simulink model "sm_car_Axle3_withDSD"  (R2022a)
settings: Solver=ode23t  StartTime=0.0  StopTime=40  MaxStep=0.4  RelTol=1e-3  AbsTol=1e-3  EnableMultiTasking=on
PreLoadFcn:
  | disp('Loading default data for 3-axle vehicle and 2-axle trailer')
  | if verLessThan('matlab', '9.11')
  |     load Vehicle_Axle3_008
  |     Vehicle = Vehicle_Axle3_008;
  |     load Trailer_Axle2_000
  |     Trailer = Trailer_Axle2_000;
  | else
  |     load Vehicle_Axle3_019
  |     Vehicle = Vehicle_Axle3_019;
  |     load Trailer_Axle2_022
  |     Trailer = Trailer_Axle2_022;
  | end
  | 
  | disp('Turning off MFEval warnings...')
  | disp('Solver:CoeffChecks:Eyk -- OFF')
  | disp('Solver:Limits:Exceeded -- OFF')
  | disp('Solver:CoeffChecks:Et -- OFF')
  | disp('Solver:CoeffChecks:Exa -- OFF')
  | 
  | warning('off','Solver:CoeffChecks:Eyk')
  | warning('off','Solver:Limits:Exceeded')
  | warning('off','Solver:CoeffChecks:Et')
  | warning('off','Solver:CoeffChecks:Exa')
  | %warning('off','Solver:Radius:NegativeRho')
  | 
  | % Due to usability issue in Repeating Sequence block
  | warning('off','Simulink:Masking:Invalid');
  | 
  | % Eliminate unnecessary warnings in inactive variants
  | % Warnings generated only if you click through inactive variant
  | warning('off','MATLAB:nonExistentField');
  | warning('off','Simulink:Parameters:BlkParamUndefined');
PostLoadFcn:
  | set_param([bdroot '/Vehicle'],'popup_trailer','On')
  | warning('off','sm:sli:setup:compile:LocalSolverNotSupported')
  | sm_car_config_maneuver(bdroot,'WOT Braking');
  | sm_car_config_vehicle(bdroot,false);
  | sm_car_config_logging(bdroot);
InitFcn:
  | sm_car_config_camera;
  | Vehicle = sm_car_vehcfg_checkConfig(Vehicle);
StartFcn:
  | sm_car_check_tire_model(bdroot);
  | tic;
StopFcn:
  | Elapsed_Sim_Time = toc;
  | % disp(['Elapsed Sim Time = ' num2str(Elapsed_Sim_Time)]);
values from neighbouring files (symbols this model uses):
  scenario = drivingScenario    [AEB_PedestrianChild_Nearside_50width_overrun.m]
undefined symbols (not defined in the file or in its folder): Maneuver, SimParams, X, Y, Z
libraries: simulink x16, Tire_Utilities x7, sm_lib x6, sm_car_DSD_lib x3, World_Config_Utilities x2, Maneuver_Get_Pose x2, Vehicle_Visualization x2, drivingscenarioandsensors x1, Camera_Frame_Definitions x1, Brake_Control x1, Driveline_Control_Axle2_None x1, Power_Control_Axle2_FixedRatio x1
(part 1 of 3)
CloseFcn:
  | try,close(h1_sm_car),end
  | clear h1_sm_car
  | try,close(h2_sm_car),end
  | clear h2_sm_car
  | try,close(h3_sm_car),end
  | clear h3_sm_car
  | try,close(h4_sm_car),end
  | clear h4_sm_car
  | 
  | 
  | clear simlog_sm_car
  | clear logsout_sm_car
Description:
  | Full Vehicle with Multibody Suspension
  | 
  | Copyright 2018-2024 The MathWorks, Inc.
settings Model: Creator=smiller  LastModifiedBy=smiller
settings SolverCC: ConcurrentTasks=on  AlgebraicLoopSolver=TrustRegion  AutoInsertRateTranBlk=on  InsertRTBMode=Never (minimum delay)
settings DataIOCC: MaxDataPoints=10000  SaveFormat=StructureWithTime  ReturnWorkspaceOutputs=off  SignalLoggingName=logsout_sm_car
settings OptimizationCC: BlockReduction=off  OptimizeBlockIOStorage=off  BufferReuse=off  GlobalBufferReuse=off  ExpressionFolding=off  LocalBlockOutputs=off  OptimizeDataStoreBuffers=off  BusAssignmentInplaceUpdate=off
settings DebuggingCC: ParameterPrecisionLossMsg=none  UnconnectedInputMsg=warning  UnconnectedOutputMsg=warning  UnconnectedLineMsg=warning  ArithmeticOperatorsInVariantConditions=warning
settings HardwareCC: ProdBitPerPointer=32  ProdBitPerSizeT=32  ProdBitPerPtrDiffT=32  ProdLargestAtomicFloat=None  ProdWordSize=32  ProdLongLongMode=on  ProdHWDeviceType=Generic->32-bit x86 compatible
settings SFSimCC: CustomCodeUndefinedFunction=UseInterfaceOnly
settings RTWCC: Description=Generic Real-Time Target  DLArmComputeVersion=19.05
settings GRTTargetCC: TargetLangStandard=C89/C90 (ANSI)
settings SimscapeCC: SimscapeLogType=all  SimscapeLogSimulationStatistics=on  SimscapeLogName=simlog_sm_car  SimscapeLogDataHistory=100000  SimscapeOperatingPoint=ssc_op
settings DiagnosticsConfigSet: SimMechanicsConflictingReferenceFrames=none  SimMechanicsRigidlyBoundBlock=none  SimMechanicsUnsatisfiedHighPriorityTargets=error
settings ExplorerConfigSet: InternalSimMechanicsExplorerSettings="<ExplorerConfiguration><canonicalview>default</canonicalview><AnimationSetting><BasePlaybackSpeed>1.0</BasePlaybackSpeed><PlaybackSpeedFactor>2.0</PlaybackSpeedFactor></AnimationSetting><TilePanel><TileInfo><Tiles Columns=\"2\" Count=\"2\" Rows=\"1\"><Column Weight=\"0.6237\"/><Column Weight=\"0.3763\"/><Row Weight=\"1\"/><Tile Height=\"1\" Width=\"1\" X=\"0\" Y=\"0\"/><Tile Height=\"1\" Width=\"1\" X=\"1\" Y=\"0\"/></Tiles></TileInfo><SceneInfo><SceneViewer><BGColor><R>1</R><G>1</G><B>1</B></BGColor><Camera><DoPerspective>on</DoPerspective><Position><X>30.8247101063582534</X><Y>0.571181504346149893</Y><Z>2.94604477699006129</Z></Position><Center><X>31.8244257672194557</X><Y>0.571174262025495705</Y><Z>2.92219949702943582</Z></Center><Up><X>0.0238451835733496931</X><Y>0.00316311256438651369</Y><Z>0.999710659110554012</Z></Up><ViewLimDist>1</ViewLimDist><YLim>0.466307658154998583</YLim><XLim>0.468997894644354318</XLim></Camera></SceneViewer><SceneViewer><BGColor><R>1</R><G>1</G><B>1</B></BGColor><Camera><DoPerspective>off</DoPerspective><Position><X>19.6858043140873598</X><Y>0.0564739167979380133</Y><Z>285.626212837348305</Z></Position><Center><X>19.6858043140873598</X><Y>0.0564739167979380133</Y><Z>2.09091177841753506</Z></Center><Up><X>0.999998132884981517</X><Y>0.0019324146943363596</Y><Z>0</Z></Up><ViewLimDist>1</ViewLimDist><YLim>18.8750577870123131</YLim><XLim>11.3976310483112808</XLim></Camera></SceneViewer></SceneInfo></TilePanel><MechEditorPanel><Cameras><Camera><Id>Camera1</Id><Value><Name>Track FixO FR</Name><NativeCamera><PositionTrackingFeature>Camera_Frames.Frame_FixO_FR.R</PositionTrackingFeature><CenterTrackingFeature>Camera_Frames.Frame_FixO_FR.R</CenterTrackingFeature><UpVectorTrackingFeature>Camera_Frames.Frame_FixO_FR.R</UpVectorTrackingFeature><CenterTrackingOrigin>off</CenterTrackingOrigin><CenterTrackingDirection>+X</CenterTrackingDirection><UpVectorTrackingDirection>+Z</UpVectorTrackingDirection></NativeCamera></Value></Camera><Camera><Id>Camera2</Id><Value><Name>Track FixO Right</Name><NativeCamera><PositionTrackingFeature>Camera_Frames.Frame_FixO_Right.R</PositionTrackingFeature><CenterTrackingFeature>Camera_Frames.Transform_Camera_Ref.F</CenterTrackingFeature><UpVectorTrackingFeature>Camera_Frames.Frame_FixO_Right.R</UpVectorTrackingFeature><CenterTrackingOrigin>off</CenterTrackingOrigin><CenterTrackingDirection>+Y</CenterTrackingDirection><UpVectorTrackingDirection>+Z</UpVectorTrackingDirection></NativeCamera></Value></Camera><Camera><Id>Camera3</Id><Value><Name>Track FixO RR</Name><NativeCamera><PositionTrackingFeature>Camera_Frames.Frame_FixO_RR.R</PositionTrackingFeature><CenterTrackingFeature>Camera_Frames.Frame_FixO_RR.R</CenterTrackingFeature><UpVectorTrackingFeature>Camera_Frames.Frame_FixO_RR.R</UpVectorTrackingFeature><CenterTrackingOrigin>off</CenterTrackingOrigin><CenterTrackingDirection>+X</CenterTrackingDirection><UpVectorTrackingDirection>+Z</UpVectorTrackingDirection></NativeCamera></Value></Camera><Camera><Id>Camera4</Id><Value><Name>Track FixO RL</Name><NativeCamera><PositionTrackingFeature>Camera_Frames.Frame_FixO_RL.R</PositionTrackingFeature><CenterTrackingFeature>Camera_Frames.Frame_FixO_RL.R</CenterTrackingFeature><UpVectorTrackingFeature>Camera_Frames.Frame_FixO_RL.R</UpVectorTrackingFeature><CenterTrackingOrigin>off</CenterTrackingOrigin><CenterTrackingDirection>+X</CenterTrackingDirection><UpVectorTrackingDirection>+Z</UpVectorTrackingDirection></NativeCamera></Value></Camera><Camera><Id>Camera5</Id><Value><Name>Track FixO Left</Name><NativeCamera><PositionTrackingFeature>Camera_Frames.Frame_FixO_Left.R</PositionTrackingFeature><CenterTrackingFeature>Camera_Frames.Transform_Camera_Ref.F</CenterTrackingFeature><UpVectorTrackingFeature>Camera_Frames.Frame_FixO_Left.R</UpVectorTrackingFeature><CenterTrackingOrigin>off</CenterTrackingOrigin><CenterTrackingDirection>-Y</CenterTrackingDirection><UpVectorTrackingDirection>+Z</UpVectorTrackingDirection></NativeCamera></Value></Camera><Camera><Id>Camera6</Id><Value><Name>Track FixO FL</Name><NativeCamera><PositionTrackingFeature>Camera_Frames.Frame_FixO_FL.R</PositionTrackingFeature><CenterTrackingFeature>Camera_Frames.Frame_FixO_FL.R</CenterTrackingFeature><UpVectorTrackingFeature>Camera_Frames.Frame_FixO_FL.R</UpVectorTrackingFeature><CenterTrackingOrigin>off</CenterTrackingOrigin><CenterTrackingDirection>+X</CenterTrackingDirection><UpVectorTrackingDirection>+Z</UpVectorTrackingDirection></NativeCamera></Value></Camera><Camera><Id>Camera7</Id><Value><Name>Track FixO Top</Name><NativeCamera><PositionTrackingFeature>Camera_Frames.Frame_FixO_Top.R</PositionTrackingFeature><CenterTrackingFeature>Camera_Frames.Frame_FixO_Top.R</CenterTrackingFeature><UpVectorTrackingFeature>Camera_Frames.Frame_FixO_Top.R</UpVectorTrackingFeature><CenterTrackingOrigin>off</CenterTrackingOrigin><CenterTrackingDirection>+X</CenterTrackingDirection><UpVectorTrackingDirection>+Z</UpVectorTrackingDirection></NativeCamera></Value></Camera><Camera><Id>Camera8</Id><Value><Name>Track FixO Front</Name><NativeCamera><PositionTrackingFeature>Camera_Frames.Frame_FixO_Front.R</PositionTrackingFeature><CenterTrackingFeature>Camera_Frames.Frame_FixO_Front.R</CenterTrackingFeature><UpVectorTrackingFeature>Camera_Frames.Frame_FixO_Front.R</UpVectorTrackingFeature><CenterTrackingOrigin>off</CenterTrackingOrigin><CenterTrackingDirection>+X</CenterTrackingDirection><UpVectorTrackingDirection>+Z</UpVectorTrackingDirection></NativeCamera></Value></Camera><Camera><Id>Camera9</Id><Value><Name>Track FixO Rear</Name><NativeCamera><PositionTrackingFeature>Camera_Frames.Frame_FixO_Rear.R</PositionTrackingFeature><CenterTrackingFeature>Camera_Frames.Frame_FixO_Rear.R</CenterTrackingFeature><UpVectorTrackingFeature>Camera_Frames.Frame_FixO_Rear.R</UpVectorTrackingFeature><CenterTrackingOrigin>off</CenterTrackingOrigin><CenterTrackingDirection>+X</CenterTrackingDirection><UpVectorTrackingDirection>+Z</UpVectorTrackingDirection></NativeCamera></Value></Camera><Camera><Id>Camera10</Id><Value><Name>Track FR</Name><NativeCamera><PositionTrackingFeature>Camera_Frames.Frame_FR.R</PositionTrackingFeature><CenterTrackingFeature>Camera_Frames.Frame_FR.R</CenterTrackingFeature><UpVectorTrackingFeature>Camera_Frames.Frame_FR.R</UpVectorTrackingFeature><CenterTrackingOrigin>off</CenterTrackingOrigin><CenterTrackingDirection>+X</CenterTrackingDirection><UpVectorTrackingDirection>+Z</UpVectorTrackingDirection></NativeCamera></Value></Camera><Camera><Id>Camera11</Id><Value><Name>Track Right</Name><NativeCamera><PositionTrackingFeature>Camera_Frames.Frame_Right.R</PositionTrackingFeature><CenterTrackingFeature>Camera_Frames.Transform_Camera_Ref.F</CenterTrackingFeature><UpVectorTrackingFeature>Camera_Frames.Frame_Right.R</UpVectorTrackingFeature><CenterTrackingOrigin>off</CenterTrackingOrigin><CenterTrackingDirection>+Y</CenterTrackingDirection><UpVectorTrackingDirection>+Z</UpVectorTrackingDirection></NativeCamera></Value></Camera><Camera><Id>Camera12</Id><Value><Name>Track RR</Name><NativeCamera><PositionTrackingFeature>Camera_Frames.Frame_RR.R</PositionTrackingFeature><CenterTrackingFeature>Camera_Frames.Frame_RR.R</CenterTrackingFeature><UpVectorTrackingFeature>Camera_Frames.Frame_RR.R</UpVectorTrackingFeature><CenterTrackingOrigin>off</CenterTrackingOrigin><CenterTrackingDirection>+X</CenterTrackingDirection><UpVectorTrackingDirection>+Z</UpVectorTrackingDirection></NativeCamera></Value></Camera><Camera><Id>Camera13</Id><Value><Name>Track RL</Name><NativeCamera><PositionTrackingFeature>Camera_Frames.Frame_RL.R</PositionTrackingFeature><CenterTrackingFeature>Camera_Frames.Frame_RL.R</CenterTrackingFeature><UpVectorTrackingFeature>Camera_Frames.Frame_RL.R</UpVectorTrackingFeature><CenterTrackingOrigin>off</CenterTrackingOrigin><CenterTrackingDirection>+X</CenterTrackingDirection><UpVectorTrackingDirection>+Z</UpVectorTrackingDirection></NativeCamera></Value></Camera><Camera><Id>Camera14</Id><Value><Name>Track Left</Name><NativeCamera><PositionTrackingFeature>Camera_Frames.Frame_Left.R</PositionTrackingFeature><CenterTrackingFeature>Camera_Frames.Transform_Camera_Ref.F</CenterTrackingFeature><UpVectorTrackingFeature>Camera_Frames.Frame_Left.R</UpVectorTrackingFeature><CenterTrackingOrigin>off</CenterTrackingOrigin><CenterTrackingDirection>-Y</CenterTrackingDirection><UpVectorTrackingDirection>+Z</UpVectorTrackingDirection></NativeCamera></Value></Camera><Camera><Id>Camera15</Id><Value><Name>Track FL</Name><NativeCamera><PositionTrackingFeature>Camera_Frames.Frame_FL.R</PositionTrackingFeature><CenterTrackingFeature>Camera_Frames.Frame_FL.R</CenterTrackingFeature><UpVectorTrackingFeature>Camera_Frames.Frame_FL.R</UpVectorTrackingFeature><CenterTrackingOrigin>off</CenterTrackingOrigin><CenterTrackingDirection>+X</CenterTrackingDirection><UpVectorTrackingDirection>+Z</UpVectorTrackingDirection></NativeCamera></Value></Camera><Camera><Id>Camera16</Id><Value><Name>Track Top</Name><NativeCamera><PositionTrackingFeature>Camera_Frames.Frame_Top.R</PositionTrackingFeature><CenterTrackingFeature>Camera_Frames.Frame_Top.R</CenterTrackingFeature><UpVectorTrackingFeature>Camera_Frames.Frame_Top.R</UpVectorTrackingFeature><CenterTrackingOrigin>off</CenterTrackingOrigin><CenterTrackingDirection>+X</CenterTrackingDirection><UpVectorTrackingDirection>+Z</UpVectorTrackingDirection></NativeCamera></Value></Camera><Camera><Id>Camera17</Id><Value><Name>Track Front</Name><NativeCamera><PositionTrackingFeature>Camera_Frames.Frame_Front.R</PositionTrackingFeature><CenterTrackingFeature>Camera_Frames.Frame_Front.R</CenterTrackingFeature><UpVectorTrackingFeature>Camera_Frames.Frame_Front.R</UpVectorTrackingFeature><CenterTrackingOrigin>off</CenterTrackingOrigin><CenterTrackingDirection>+X</CenterTrackingDirection><UpVectorTrackingDirection>+Z</UpVectorTrackingDirection></NativeCamera></Value></Camera><Camera><Id>Camera18</Id><Value><Name>Track Rear</Name><NativeCamera><PositionTrackingFeature>Camera_Frames.Frame_Rear.R</PositionTrackingFeature><CenterTrackingFeature>Camera_Frames.Frame_Rear.R</CenterTrackingFeature><UpVectorTrackingFeature>Camera_Frames.Frame_Rear.R</UpVectorTrackingFeature><CenterTrackingOrigin>off</CenterTrackingOrigin><CenterTrackingDirection>+X</CenterTrackingDirection><UpVectorTrackingDirection>+Z</UpVectorTrackingDirection></NativeCamera></Value></Camera><Camera><Id>Camera19</Id><Value><Name>Track SuspF</Name><NativeCamera><PositionTrackingFeature>Camera_Frames.Frame_SuspF.R</PositionTrackingFeature><CenterTrackingFeature>Camera_Frames.Frame_SuspF.R</CenterTrackingFeature><UpVectorTrackingFeature>Camera_Frames.Frame_SuspF.R</UpVectorTrackingFeature><CenterTrackingOrigin>off</CenterTrackingOrigin><CenterTrackingDirection>+X</CenterTrackingDirection><UpVectorTrackingDirection>+Z</UpVectorTrackingDirection></NativeCamera></Value></Camera><Camera><Id>Camera20</Id><Value><Name>Track SuspR</Name><NativeCamera><PositionTrackingFeature>Camera_Frames.Frame_SuspR.R</PositionTrackingFeature><CenterTrackingFeature>Camera_Frames.Frame_SuspR.R</CenterTrackingFeature><UpVectorTrackingFeature>Camera_Frames.Frame_SuspR.R</UpVectorTrackingFeature><CenterTrackingOrigin>off</CenterTrackingOrigin><CenterTrackingDirection>+X</CenterTrackingDirection><UpVectorTrackingDirection>+Z</UpVectorTrackingDirection></NativeCamera></Value></Camera><Camera><Id>Camera21</Id><Value><Name>Track WheelFR</Name><NativeCamera><PositionTrackingFeature>Camera_Frames.Frame_Wheel_FR.R</PositionTrackingFeature><CenterTrackingFeature>Camera_Frames.Frame_Wheel_FR.R</CenterTrackingFeature><UpVectorTrackingFeature>Camera_Frames.Frame_Wheel_FR.R</UpVectorTrackingFeature><CenterTrackingOrigin>off</CenterTrackingOrigin><CenterTrackingDirection>+X</CenterTrackingDirection><UpVectorTrackingDirection>+Z</UpVectorTrackingDirection></NativeCamera></Value></Camera><Camera><Id>Camera22</Id><Value><Name>Track WheelRR</Name><NativeCamera><PositionTrackingFeature>Camera_Frames.Frame_Wheel_RR.R</PositionTrackingFeature><CenterTrackingFeature>Camera_Frames.Frame_Wheel_RR.R</CenterTrackingFeature><UpVectorTrackingFeature>Camera_Frames.Frame_Wheel_RR.R</UpVectorTrackingFeature><CenterTrackingOrigin>off</CenterTrackingOrigin><CenterTrackingDirection>+X</CenterTrackingDirection><UpVectorTrackingDirection>+Z</UpVectorTrackingDirection></NativeCamera></Value></Camera><Camera><Id>Camera23</Id><Value><Name>Track WheelRL</Name><NativeCamera><PositionTrackingFeature>Camera_Frames.Frame_Wheel_RL.R</PositionTrackingFeature><CenterTrackingFeature>Camera_Frames.Frame_Wheel_RL.R</CenterTrackingFeature><UpVectorTrackingFeature>Camera_Frames.Frame_Wheel_RL.R</UpVectorTrackingFeature><CenterTrackingOrigin>off</CenterTrackingOrigin><CenterTrackingDirection>+X</CenterTrackingDirection><UpVectorTrackingDirection>+Z</UpVectorTrackingDirection></NativeCamera></Value></Camera><Camera><Id>Camera24</Id><Value><Name>Track WheelFL</Name><NativeCamera><PositionTrackingFeature>Camera_Frames.Frame_Wheel_FL.R</PositionTrackingFeature><CenterTrackingFeature>Camera_Frames.Frame_Wheel_FL.R</CenterTrackingFeature><UpVectorTrackingFeature>Camera_Frames.Frame_Wheel_FL.R</UpVectorTrackingFeature><CenterTrackingOrigin>off</CenterTrackingOrigin><CenterTrackingDirection>+X</CenterTrackingDirection><UpVectorTrackingDirection>+Z</UpVectorTrackingDirection></NativeCamera></Value></Camera><Camera><Id>Camera25</Id><Value><Name>View Seat FL</Name><NativeCamera><PositionTrackingFeature>Camera_Frames.Frame_View_Seat_FL.R</PositionTrackingFeature><CenterTrackingFeature>Camera_Frames.Frame_View_Seat_FL.R</CenterTrackingFeature><UpVectorTrackingFeature>Camera_Frames.Frame_View_Seat_FL.R</UpVectorTrackingFeature><CenterTrackingOrigin>off</CenterTrackingOrigin><CenterTrackingDirection>+X</CenterTrackingDirection><UpVectorTrackingDirection>+Z</UpVectorTrackingDirection></NativeCamera></Value></Camera><Camera><Id>Camera26</Id><Value><Name>View Seat FR</Name><NativeCamera><PositionTrackingFeature>Camera_Frames.Frame_View_Seat_FR.R</PositionTrackingFeature><CenterTrackingFeature>Camera_Frames.Frame_View_Seat_FR.R</CenterTrackingFeature><UpVectorTrackingFeature>Camera_Frames.Frame_View_Seat_FR.R</UpVectorTrackingFeature><CenterTrackingOrigin>off</CenterTrackingOrigin><CenterTrackingDirection>+X</CenterTrackingDirection><UpVectorTrackingDirection>+Z</UpVectorTrackingDirection></NativeCamera></Value></Camera><Camera><Id>Camera27</Id><Value><Name>View Susp FR</Name><NativeCamera><PositionTrackingFeature>Camera_Frames.Frame_View_Susp_FR.R</PositionTrackingFeature><CenterTrackingFeature>Camera_Frames.Frame_View_Susp_FR.R</CenterTrackingFeature><UpVectorTrackingFeature>Camera_Frames.Frame_View_Susp_FR.R</UpVectorTrackingFeature><CenterTrackingOrigin>off</CenterTrackingOrigin><CenterTrackingDirection>+X</CenterTrackingDirection><UpVectorTrackingDirection>+Z</UpVectorTrackingDirection></NativeCamera></Value></Camera><Camera><Id>Camera28</Id><Value><Name>View Susp RR</Name><NativeCamera><PositionTrackingFeature>Camera_Frames.Frame_View_Susp_RR.R</PositionTrackingFeature><CenterTrackingFeature>Camera_Frames.Frame_View_Susp_RR.R</CenterTrackingFeature><UpVectorTrackingFeature>Camera_Frames.Frame_View_Susp_RR.R</UpVectorTrackingFeature><CenterTrackingOrigin>off</CenterTrackingOrigin><CenterTrackingDirection>+X</CenterTrackingDirection><UpVectorTrackingDirection>+Z</UpVectorTrackingDirection></NativeCamera></Value></Camera><Camera><Id>Camera29</Id><Value><Name>View Susp RL</Name><NativeCamera><PositionTrackingFeature>Camera_Frames.Frame_View_Susp_RL.R</PositionTrackingFeature><CenterTrackingFeature>Camera_Frames.Frame_View_Susp_RL.R</CenterTrackingFeature><UpVectorTrackingFeature>Camera_Frames.Frame_View_Susp_RL.R</UpVectorTrackingFeature><CenterTrackingOrigin>off</CenterTrackingOrigin><CenterTrackingDirection>+X</CenterTrackingDirection><UpVectorTrackingDirection>+Z</UpVectorTrackingDirection></NativeCamera></Value></Camera><Camera><Id>Camera30</Id><Value><Name>View Susp FL</Name><NativeCamera><PositionTrackingFeature>Camera_Frames.Frame_View_Susp_FL.R</PositionTrackingFeature><CenterTrackingFeature>Camera_Frames.Frame_View_Susp_FL.R</CenterTrackingFeature><UpVectorTrackingFeature>Camera_Frames.Frame_View_Susp_FL.R</UpVectorTrackingFeature><CenterTrackingOrigin>off</CenterTrackingOrigin><CenterTrackingDirection>+X</CenterTrackingDirection><UpVectorTrackingDirection>+Z</UpVectorTrackingDirection></NativeCamera></Value></Camera><Camera><Id>Camera31</Id><Value><Name>Dolly Camera</Name><NativeCamera><PositionTrackingFeature>Camera_Frames.Frame_Dolly.R</PositionTrackingFeature><CenterTrackingFeature>Camera_Frames.Frame_Dolly.R</CenterTrackingFeature><UpVectorTrackingFeature>Camera_Frames.Frame_Dolly.R</UpVectorTrackingFeature><CenterTrackingOrigin>off</CenterTrackingOrigin><CenterTrackingDirection>+X</CenterTrackingDirection><UpVectorTrackingDirection>+Z</UpVectorTrackingDirection></NativeCamera></Value></Camera><Camera><Id>Camera32</Id><Value><Name>Track Dolly Camera</Name><NativeCamera><PositionTrackingFeature>Camera_Frames.Frame_Dolly.R</PositionTrackingFeature><CenterTrackingFeature>Camera_Frames.Transform_Camera_Ref.F</CenterTrackingFeature><UpVectorTrackingFeature>Camera_Frames.World_Frame.W</UpVectorTrackingFeature><CenterTrackingOrigin>on</CenterTrackingOrigin><UpVectorTrackingDirection>+Z</UpVectorTrackingDirection></NativeCamera></Value></Camera></Cameras><GfxPanelCameraMap><MapElement CameraMLId=\"Camera25\" GfxPanelIndex=\"0\"/></GfxPanelCameraMap><VideoCreator><PlaybackSpeedRatio>1.0</PlaybackSpeedRatio><FrameRate>30</FrameRate><VideoFormat>MPEG-4</VideoFormat><FrameSize>[800 450]</FrameSize></VideoCreator></MechEditorPanel></ExplorerConfiguration>"

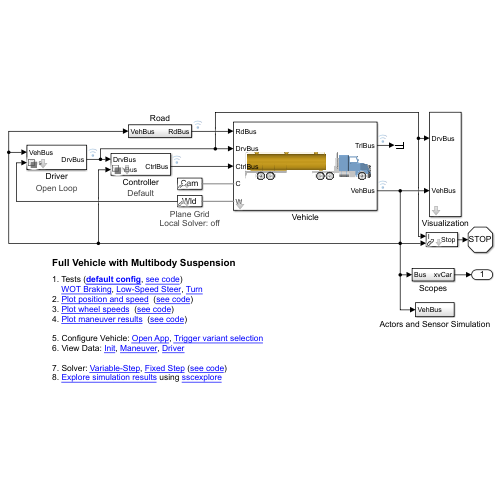
[thumbnail: Simulink's stored preview of the top-level diagram]
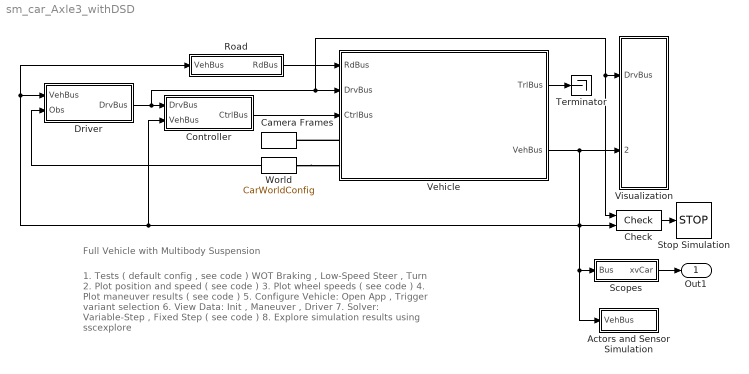
== system sm_car_Axle3_withDSD ==
  note: Full Vehicle with Multibody Suspension
  note: 1. Tests ( default config , see code )
      | WOT Braking , Low-Speed Steer , Turn
      | 2. Plot position and speed ( see code )
      | 3. Plot wheel speeds ( see code )
      | 4. Plot maneuver results ( see code )
      |
      | 5. Configure Vehicle: Open App , Trigger variant selection
      | 6. View Data: Init , Maneuver , Driver
      |
      | 7. Solver: Variable-Step , Fixed Step ( see code )
      | 8. Explore simulation results using sscexplore
  Actors and Sensor Simulation : Subsystem
  Camera Frames : Camera_Frame_Definitions/Camera Frames  Camera=Camera  popup_dolly_camera=Off
  Check : World_Config_Utilities/Check  stop_speed=0.1  start_check_time=5  max_speed=0.4  start_check_time_max_speed=20000  lat_dev_threshold=8  start_check_time_ld=10000  end_lap_num=1  start_check_time_end_lap=10000  max_dist_threshold=10000  start_check_time_max_dist=10000
  Controller : Subsystem  Variant=on  VariantControlMode=label  VariantControl=Variant1  LabelModeActiveChoice=Default  mask{popup_control=Default}
      mask prompts: popup_control "Control"
      mask init:
      | temp_ctrlMode = get_param(gcb,'popup_control');
      | if(strcmp(temp_ctrlMode,'Default'))
      |     set_param(gcb,'LabelModeActiveChoice','Default');
      | elseif(strcmp(temp_ctrlMode,'Fuel Cell 1 Motor'))
      |     set_param(gcb,'LabelModeActiveChoice','FuelCell1Motor');
      | end
      settings: AttributesFormatString=%<popup_control>
      mask TypeOptions popup_control: Default
      mask Display: disp(' ');
  Driver : Subsystem  Variant=on  VariantControlMode=label  VariantControl=Variant1  LabelModeActiveChoice=Open_Loop  mask{popup_driver_type=Open Loop}
      mask prompts: popup_driver_type "Driver"
      mask init:
      | set_param(gcb,'LabelModeActiveChoice',strrep(get_param(gcb,'popup_driver_type'),' ','_'));
      settings: AttributesFormatString=%<popup_driver_type>
      mask TypeOptions popup_driver_type: Open Loop | Drive Cycle | Closed Loop | Interactive
      mask Display: disp(' ')
  Road : Subsystem
  Scopes : Subsystem
  Stop Simulation : Stop
  Terminator : Terminator
  Vehicle : Subsystem  mask{popup_trailer=On}
      mask prompts: popup_trailer "Trailer"
      mask init:
      | if(strcmp(get_param(gcb,'popup_trailer'),'On'))
      |     set_param([gcb '/Trailer'],'LabelModeActiveChoice','Trailer');
      |     set_param([gcb '/Hitch'],'LabelModeActiveChoice','On');
      | else
      |     set_param([gcb '/Trailer'],'LabelModeActiveChoice','None');
      |     set_param([gcb '/Hitch'],'LabelModeActiveChoice','Off');
      | end
      mask TypeOptions popup_trailer: On | Off
      mask Display:
      | % Assemble image from BodyGeometry.class
      | % (active choice from Body Geometry subsystem)
      | 
      | temp_trl_bg_class = 'none';
      | if(strcmp(get_param(gcb,'popup_trailer'),'On'))
      |     temp_trl_bg_class = lower(get_param([gcb '/Trailer/Trailer/Chassis/Body/Body Geometry'],'LabelModeActiveChoice'));
      | end
      | temp_veh_bg_class = lower(get_param([gcb '/Vehicle/Chassis/Body/Body Geometry'],'LabelModeActiveChoice'));
      | 
      | % Same body geometry used for 2-axle and 3-axle busses
      | % 3-axle image used here
      | temp_veh_bg_class = strrep(temp_veh_bg_class,'_makhulu','_makhulu3axle');
      | 
      | imagestr = (['sm_car_vehicle_' temp_veh_bg_class '_' temp_trl_bg_class '.png']);
      | 
      | % If image does not exist, use default image
      | % Changes based on trailer popup
      | if(~exist(imagestr))
      |     if(strcmp(get_param(gcb,'popup_trailer'),'On'))
      |         temp_trl_bg_class = 'default';
      |     else
      |         temp_trl_bg_class = 'none';
      |     end
      |     imagestr = ['sm_car_vehicle_axle3_default_' temp_trl_bg_class '.png'];
      | end
      | 
      | image(imagestr);
  Visualization : Subsystem  mask{unreal_onoff=Off}
      mask prompts: unreal_onoff "Unreal Animation"
      mask init:
      | set_param([gcb '/Unreal'],'popup_animation',get_param(gcb,'unreal_onoff'));
      mask TypeOptions unreal_onoff: Off | On
  World : World_Config_Utilities/CarWorldConfig  UseLocalSolver=off  LocalSolverChoice=Backward Euler  LocalSolverSampleTime=0.005  DoFixedCost=off  MaxNonlinIter=3  popup_scene=Plane Grid  popup_gravity=Constant  GravityVector=[0 0 -9.80665]
      settings: AttributesFormatString=|
      | %<popup_scene>
      | Local Solver: %<UseLocalSolver>
  Out1 : Outport  VectorParamsAs1DForOutWhenUnconnected=off
  wires:
  Check/1 -> Stop Simulation/1
  Scopes/1(xvCar) -> Out1/1
  Driver/1(" DrvBus") -> Controller/1("DrvBus "), Check/1, Visualization/1(DrvBus), Vehicle/2(DrvBus)
  Vehicle/2(VehBus) -> Visualization/2(VehBus), Actors and Sensor Simulation/1(VehBus), Scopes/1(Bus), Controller/2("VehBus "), Driver/1("VehBus "), Road/1(VehBus), Check/2
  Road/1(RdBus) -> Vehicle/1(RdBus)
  Controller/1(" CtrlBus") -> Vehicle/3(CtrlBus)
  Vehicle/1(TrlBus) -> Terminator/1
  World/1 -> Driver/2(Obs)
  connections:
  Vehicle/LConn1 -- Camera Frames/RConn1
  World/LConn1 -- Vehicle/LConn2

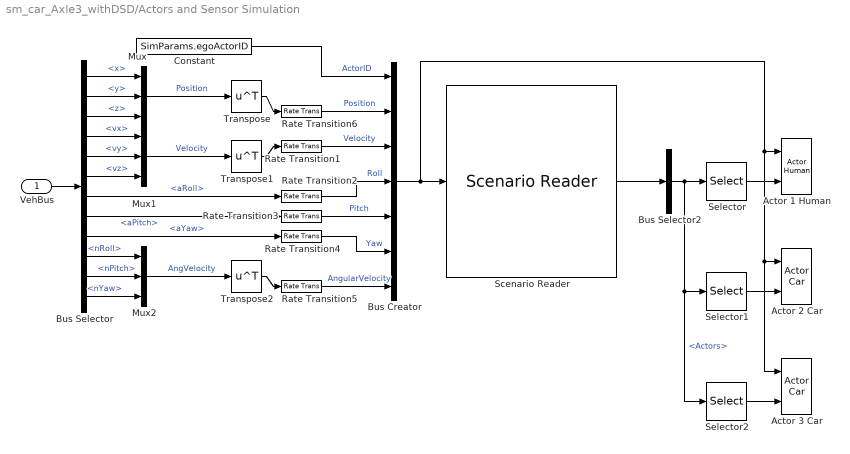
== system sm_car_Axle3_withDSD/Actors and Sensor Simulation ==
  VehBus : Inport
  Actor 1 Human : sm_car_DSD_lib/Actor Human  SystemSampleTime=-1  VariantActivationTime=update diagram  Latency=0  AutoFrameSizeCalculation=off
  Actor 2 Car : sm_car_DSD_lib/Actor Car  car_track=scenario.Actors(1,2).Width  clr_body_geo_left=scenario.Actors(1,2).PlotColor  whl_base=scenario.Actors(1,2).Wheelbase  offset_ref=[1.5 0 0.3225]  opc_body_geo_left=0.5
  Actor 3 Car : sm_car_DSD_lib/Actor Car  car_track=scenario.Actors(1,3).Width  clr_body_geo_left=scenario.Actors(1,3).PlotColor  whl_base=scenario.Actors(1,3).Wheelbase  offset_ref=[1.5 0 0.3225]  opc_body_geo_left=0.5
  Bus Creator : BusCreator  Inputs=7  OutDataTypeStr=Bus: BusActorsActors  NonVirtualBus=on
  Bus Selector : BusSelector  OutputSignals=World.x,World.y,World.z,World.vx,World.vy,World.vz,World.aRoll,World.aPitch,World.aYaw,World.nRoll,World.nPitch,World.nYaw
  Bus Selector2 : BusSelector  OutputSignals=Actors
  Constant : Constant  Value=SimParams.egoActorID
  Mux : Mux  Inputs=3
  Mux1 : Mux  Inputs=3
  Mux2 : Mux  Inputs=3
  Rate Transition{1..6} (6 alike) : RateTransition  OutPortSampleTime=SimParams.Ts
  Scenario Reader : drivingscenarioandsensors/Scenario Reader  ScenarioSource=From workspace  ScenarioFileName=AEB_CCRs_100overlap.mat  ScenarioVariableName=scenario  OutputCoordinateSystem=Vehicle coordinates  EgoVehicleSource=Input port  EgoVehicleActorID=SimParams.egoActorID  OrientVehiclesOnRoad=off  OutputEgoVehiclePose=off  OutputEgoVehicleState=off  SampleTime=SimParams.Ts  LaneBoundaryOutput=None  LaneBoundaryDistance=0:0.5:9.5  LaneBoundaryLocation=Center of lane markings  BusNameSource=Property  BusName=busActors  BusNumActorsSource=Scenario  BusNumActors=100  BusName2Source=Auto  BusName2=BusLaneBoundaries  BusNumLaneBoundariesSource=Scenario  BusNumLaneBoundaries=10  BusName3Source=Auto  BusName3=BusEgoActor  BusName4Source=Auto  BusName4=BusEgoState  ShowCoordinateLabels=on  SimulateUsing=Interpreted execution
  Selector : Selector  InputPortWidth=3  IndexOptions=Index vector (dialog)  Indices=1  OutputSizes=1
  Selector1 : Selector  InputPortWidth=3  IndexOptions=Index vector (dialog)  Indices=2  OutputSizes=1
  Selector2 : Selector  InputPortWidth=3  IndexOptions=Index vector (dialog)  Indices=3  OutputSizes=1
  Transpose : Math  Operator=transpose
  Transpose1 : Math  Operator=transpose
  Transpose2 : Math  Operator=transpose
  wires:
  VehBus/1 -> Bus Selector/1
  Rate Transition6/1 -> Bus Creator/2  "Position"
  Bus Selector/1 -> Mux/1  "<x>"
  Bus Selector/2 -> Mux/2  "<y>"
  Bus Selector/3 -> Mux/3  "<z>"
  Bus Selector/4 -> Mux1/1  "<vx>"
  Bus Selector/5 -> Mux1/2  "<vy>"
  Bus Selector/6 -> Mux1/3  "<vz>"
  Rate Transition1/1 -> Bus Creator/3  "Velocity"
  Rate Transition2/1 -> Bus Creator/4  "Roll"
  Mux/1 -> Transpose/1  "Position"
  Mux1/1 -> Transpose1/1  "Velocity"
  Bus Selector/7 -> Rate Transition2/1  "<aRoll>"
  Bus Selector/8 -> Rate Transition3/1  "<aPitch>"
  Rate Transition3/1 -> Bus Creator/5  "Pitch"
  Bus Selector/9 -> Rate Transition4/1  "<aYaw>"
  Rate Transition4/1 -> Bus Creator/6  "Yaw"
  Bus Selector/10 -> Mux2/1  "<nRoll>"
  Bus Selector/11 -> Mux2/2  "<nPitch>"
  Bus Selector/12 -> Mux2/3  "<nYaw>"
  Mux2/1 -> Transpose2/1  "AngVelocity"
  Rate Transition5/1 -> Bus Creator/7  "AngularVelocity"
  Constant/1 -> Bus Creator/1  "ActorID"
  Bus Creator/1 -> Actor 1 Human/1, Actor 3 Car/1, Actor 2 Car/1, Scenario Reader/1
  Transpose/1 -> Rate Transition6/1
  Transpose1/1 -> Rate Transition1/1
  Transpose2/1 -> Rate Transition5/1
  Selector/1 -> Actor 1 Human/2
  Selector1/1 -> Actor 2 Car/2
  Selector2/1 -> Actor 3 Car/2
  Bus Selector2/1 -> Selector2/1, Selector1/1, Selector/1  "<Actors>"
  Scenario Reader/1 -> Bus Selector2/1

== system sm_car_Axle3_withDSD/Controller ==
  "DrvBus " : Inport
  "VehBus " : Inport  Port=2
  Default : Subsystem  VariantControl=Default
  " CtrlBus" : Outport  VectorParamsAs1DForOutWhenUnconnected=off

== system sm_car_Axle3_withDSD/Driver ==
  "VehBus " : Inport
  Obs : Inport  Port=2
  Closed Loop : Subsystem  VariantControl=Closed_Loop
  Drive Cycle : Driver_Drive_Cycle/Drive Cycle  SystemSampleTime=-1  VariantControl=Drive_Cycle  VariantActivationTime=update diagram  Latency=0  AutoFrameSizeCalculation=off
  Interactive : Subsystem  VariantControl=Interactive  mask{popup_pace_car=None}
      mask prompts: popup_pace_car "Pace Car"
      mask init:
      | set_param([gcb '/Pace Car'],'popup_pace_car',get_param(gcb,'popup_pace_car'));
      settings: AttributesFormatString=Pace Car: %<popup_pace_car>
      mask TypeOptions popup_pace_car: None | Show
  Open Loop : Subsystem  VariantControl=Open_Loop
  " DrvBus" : Outport  VectorParamsAs1DForOutWhenUnconnected=off

== system sm_car_Axle3_withDSD/Road ==
  VehBus : Inport
  Bus Creator : BusCreator  Inputs=8
  Bus Selector1 : BusSelector  OutputSignals=Chassis
  Ground : Tire_Utilities/Ground Axle3  SystemSampleTime=-1  VariantActivationTime=update diagram  Latency=0  AutoFrameSizeCalculation=off
  Input fWindCar : Subsystem  mask{fWind=[0 0 0], tWind=2, dWind=30000}
      mask prompts: fWind "Force [x y z] (N)"; tWind "Duration (s)"; dWind "Start time (sec)"
  Input fWindTrailer : Subsystem  mask{fWind=[0 0 0], tWind=2, dWind=30000}
      mask prompts: fWind "Force [x y z] (N)"; tWind "Duration (s)"; dWind "Start time (sec)"
  Mu Scaling by Position : Subsystem  mask{muFL_out=1, muFR_out=1, muRL_out=1, muRR_out=1, muFL_in=1, muFR_in=1, muRL_in=1, muRR_in=1, intvX_FL_start=100-40, intvX_FR_start=100-40, intvX_RL_start=100-40, intvX_RR_start=100-40, intvX_FL_end=130-40, intvX_FR_end=130-40, intvX_RL_end=130-40, intvX_RR_end=130-40, intvY_FL_start=-30, intvY_FR_start=-30, intvY_RL_start=-30, intvY_RR_start=-30, intvY_FL_end=0, intvY_FR_end=0, intvY_RL_end=0, intvY_RR_end=0}
      mask TypeOptions muFL_out: muL1 out/Value
      mask TypeOptions muFR_out: muR1 out/Value
      mask TypeOptions muRL_out: muL2 out/Value
      mask TypeOptions muRR_out: muR2 out/Value
      mask TypeOptions muFL_in: muL 1in/Value
      mask TypeOptions muFR_in: muR1 in/Value
      mask TypeOptions muRL_in: muL2 in/Value
      mask TypeOptions muRR_in: muR2 in/Value
      mask TypeOptions intvX_FL_start: Interval Test L1x/lowlimit
      mask TypeOptions intvX_FR_start: Interval Test R1x/lowlimit
      mask TypeOptions intvX_RL_start: Interval Test L2x/lowlimit
      mask TypeOptions intvX_RR_start: Interval Test R2x/lowlimit
      mask TypeOptions intvX_FL_end: Interval Test L1x/uplimit
      mask TypeOptions intvX_FR_end: Interval Test R1x/uplimit
      mask TypeOptions intvX_RL_end: Interval Test L2x/uplimit
      mask TypeOptions intvX_RR_end: Interval Test R2x/uplimit
      mask TypeOptions intvY_FL_start: Interval Test L1y/lowlimit
      mask TypeOptions intvY_FR_start: Interval Test R1y/lowlimit
      mask TypeOptions intvY_RL_start: Interval Test L2y/lowlimit
      mask TypeOptions intvY_RR_start: Interval Test R2y/lowlimit
      mask TypeOptions intvY_FL_end: Interval Test L1y/uplimit
      mask TypeOptions intvY_FR_end: Interval Test R1y/uplimit
      mask TypeOptions intvY_RL_end: Interval Test L2y/uplimit
      mask TypeOptions intvY_RR_end: Interval Test R2y/uplimit
      mask DialogControl text_whl Prompt: Wheel
      mask DialogControl text_FL Prompt: FL
      mask DialogControl text_FR Prompt: FR
      mask DialogControl text_RL Prompt: RL
      mask DialogControl text_RR Prompt: RR
      mask DialogControl text_mu Prompt: mu
      mask DialogControl text_mu_intv Prompt: mu intv
      mask DialogControl text_x_start Prompt: X Start (m)
      mask DialogControl text_x_end Prompt: X End (m)
      mask DialogControl text_y_start Prompt: Y Start (m)
      mask DialogControl text_y_end Prompt: Y End (m)
  Road Surface Height : Surface_Profile_Axle3/Road Surface Profile Axle3  LabelModeActiveChoice=None
      settings: AttributesFormatString=%<LabelModeActiveChoice>
  RdBus : Outport  VectorParamsAs1DForOutWhenUnconnected=off
  wires:
  VehBus/1 -> Bus Selector1/1
  Mu Scaling by Position/1(L1) -> Ground/3
  Bus Selector1/1 -> Road Surface Height/1, Mu Scaling by Position/1(Chassis)  "<Chassis>"
  Mu Scaling by Position/4(R2) -> Ground/6
  Road Surface Height/1 -> Ground/1
  Mu Scaling by Position/3(L2) -> Ground/5
  Bus Creator/1 -> RdBus/1  "RdBus"
  Mu Scaling by Position/2(R1) -> Ground/4
  Ground/1 -> Bus Creator/1
  Ground/2 -> Bus Creator/2
  Ground/3 -> Bus Creator/3
  Ground/4 -> Bus Creator/4
  Input fWindCar/1(fWind) -> Bus Creator/7  "fWindCar"
  Input fWindTrailer/1(fWind) -> Bus Creator/8  "fWindTrailer"
  Road Surface Height/2 -> Ground/2
  Ground/5 -> Bus Creator/5
  Ground/6 -> Bus Creator/6
  Mu Scaling by Position/5(L3) -> Ground/7
  Mu Scaling by Position/6(R3) -> Ground/8

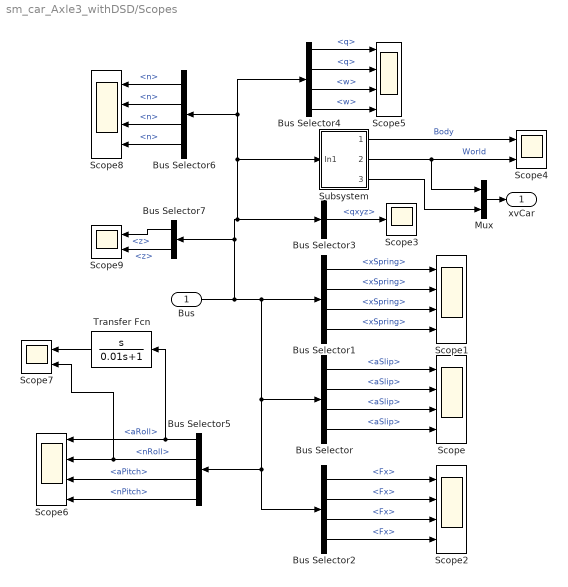
== system sm_car_Axle3_withDSD/Scopes ==
  Bus : Inport
  Bus Selector : BusSelector  OutputSignals=Chassis.WhlL1.aSlip,Chassis.WhlR1.aSlip,Chassis.WhlL2.aSlip,Chassis.WhlR2.aSlip
  Bus Selector1 : BusSelector  OutputSignals=Chassis.Spring.L1.xSpring,Chassis.Spring.R1.xSpring,Chassis.Spring.L2.xSpring,Chassis.Spring.R2.xSpring
  Bus Selector2 : BusSelector  OutputSignals=Chassis.WhlL1.Fx,Chassis.WhlR1.Fx,Chassis.WhlL2.Fx,Chassis.WhlR2.Fx
  Bus Selector3 : BusSelector  OutputSignals=Chassis.WhlL1.qxyz
  Bus Selector4 : BusSelector  OutputSignals=Driveline.anDriveshaftL1.q,Driveline.anDriveshaftR1.q,Driveline.anDriveshaftL1.w,Driveline.anDriveshaftR1.w
  Bus Selector5 : BusSelector  OutputSignals=Chassis.Body.CG.aRoll,Chassis.Body.CG.nRoll,Chassis.Body.CG.aPitch,Chassis.Body.CG.nPitch
  Bus Selector6 : BusSelector  OutputSignals=Chassis.WhlL1.n,Chassis.WhlR1.n,Chassis.WhlR2.n,Chassis.WhlL2.n
  Bus Selector7 : BusSelector  OutputSignals=Chassis.Body.CG.z,World.z
  Mux : Mux  Inputs=2
  Scope{,1..2,5..6,8} (6 alike) : Scope  NumInputPorts=4
  Scope3 : Scope
  Scope4 : Scope  NumInputPorts=2
  Scope7 : Scope  NumInputPorts=2
  Scope9 : Scope  NumInputPorts=2
  Subsystem : Subsystem
  Transfer Fcn : TransferFcn  Numerator=[1 0]  Denominator=[0.01 1]
  xvCar : Outport  VectorParamsAs1DForOutWhenUnconnected=off
  wires:
  Bus/1 -> Bus Selector1/1, Bus Selector2/1, Bus Selector5/1, Bus Selector/1, Bus Selector7/1, Subsystem/1(In1), Bus Selector6/1, Bus Selector4/1, Bus Selector3/1
  Bus Selector/1 -> Scope/1  "<aSlip>"
  Bus Selector/2 -> Scope/2  "<aSlip>"
  Bus Selector/3 -> Scope/3  "<aSlip>"
  Bus Selector/4 -> Scope/4  "<aSlip>"
  Bus Selector1/1 -> Scope1/1  "<xSpring>"
  Bus Selector1/2 -> Scope1/2  "<xSpring>"
  Bus Selector1/3 -> Scope1/3  "<xSpring>"
  Bus Selector1/4 -> Scope1/4  "<xSpring>"
  Bus Selector2/3 -> Scope2/3  "<Fx>"
  Bus Selector2/4 -> Scope2/4  "<Fx>"
  Bus Selector2/2 -> Scope2/2  "<Fx>"
  Bus Selector2/1 -> Scope2/1  "<Fx>"
  Bus Selector3/1 -> Scope3/1  "<qxyz>"
  Subsystem/1(vBody) -> Scope4/1  "Body"
  Subsystem/2(vWorld) -> Mux/1, Scope4/2  "World"
  Mux/1 -> xvCar/1
  Subsystem/3(xWorld) -> Mux/2
  Bus Selector4/2 -> Scope5/2  "<q>"
  Bus Selector4/1 -> Scope5/1  "<q>"
  Bus Selector4/3 -> Scope5/3  "<w>"
  Bus Selector4/4 -> Scope5/4  "<w>"
  Bus Selector5/1 -> Scope6/1, Transfer Fcn/1  "<aRoll>"
  Bus Selector5/2 -> Scope7/2, Scope6/2  "<nRoll>"
  Bus Selector5/3 -> Scope6/3  "<aPitch>"
  Bus Selector5/4 -> Scope6/4  "<nPitch>"
  Transfer Fcn/1 -> Scope7/1
  Bus Selector6/1 -> Scope8/1  "<n>"
  Bus Selector6/2 -> Scope8/2  "<n>"
  Bus Selector6/3 -> Scope8/3  "<n>"
  Bus Selector6/4 -> Scope8/4  "<n>"
  Bus Selector7/1 -> Scope9/1  "<z>"
  Bus Selector7/2 -> Scope9/2  "<z>"

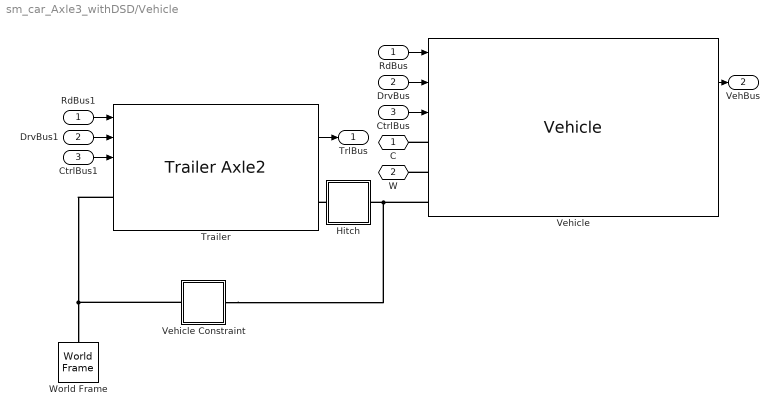
== system sm_car_Axle3_withDSD/Vehicle ==
  RdBus : Inport
  DrvBus : Inport  Port=2
  CtrlBus : Inport  Port=3
  CtrlBus1 : InportShadow  Port=3
  DrvBus1 : InportShadow  Port=2
  Hitch : Subsystem  Variant=on  VariantControlMode=label  VariantControl=Variant1  LabelModeActiveChoice=On  mask(Hitch Connection){}
      mask help: Set to "On" if Trailer is present.
      settings: AttributesFormatString=%<LabelModeActiveChoice>
      mask Display: disp(' ');
  RdBus1 : InportShadow
  Trailer : Trailer_Axle2/Trailer Axle2  VariantControl=NS_Con  LabelModeActiveChoice=Trailer  veh_index=41  SpecifyPosTarget=off
      settings: AttributesFormatString=%<LabelModeActiveChoice>
  Vehicle : Vehicle_Axle3/Vehicle  Tag=PublishSubsystem  VariantControl=NS_Con  popup_wheel_spin=Free  popup_BodyToWorld=Free  Vehicle=Vehicle  Init=Init  veh_index=1  mask_image_name=sm_car_vehicle_hambalg_IMAGE.png
  Vehicle Constraint : Subsystem  Variant=on  VariantControlMode=label  VariantControl=Choice  LabelModeActiveChoice=NoConstraint
      settings: AttributesFormatString=%<LabelModeActiveChoice>
      mask Display: disp(' ');
  World Frame : sm_lib/Frames and Transforms/World Frame
  C : PMIOPort  Side=Left
  W : PMIOPort  Port=2  Side=Left
  TrlBus : Outport  VectorParamsAs1DForOutWhenUnconnected=off
  VehBus : Outport  Port=2  VectorParamsAs1DForOutWhenUnconnected=off
  wires:
  DrvBus/1 -> Vehicle/2
  CtrlBus/1 -> Vehicle/3
  Vehicle/1 -> VehBus/1
  RdBus/1 -> Vehicle/1
  RdBus1/1 -> Trailer/1
  DrvBus1/1 -> Trailer/2
  CtrlBus1/1 -> Trailer/3
  Trailer/1 -> TrlBus/1
  connections:
  Vehicle/LConn1 -- C/RConn1
  Vehicle/LConn2 -- W/RConn1
  Trailer/LConn2 -- Vehicle Constraint/LConn1 -- World Frame/RConn1
  Vehicle/LConn3 -- Vehicle Constraint/RConn1 -- Hitch/LConn1
  Hitch/RConn1 -- Trailer/RConn1

== system sm_car_Axle3_withDSD/Visualization ==
  DrvBus : Inport
  VehBus : Inport  Port=2
  Bus Creator : BusCreator  Inputs=5
  Dashboard : Subsystem
  Data for Unreal : Vehicle_Visualization/Data for Unreal  SystemSampleTime=-1  VariantActivationTime=update diagram  Latency=0  AutoFrameSizeCalculation=off
  Terminator : Terminator
  Unreal : Subsystem  Variant=on  VariantControlMode=label  VariantControl=Variant1  LabelModeActiveChoice=Off  mask{popup_animation=Off}
      mask prompts: popup_animation "Animation"
      mask init:
      | set_param(gcb,'LabelModeActiveChoice',get_param(gcb,'popup_animation'));
      settings: AttributesFormatString=%<LabelModeActiveChoice>
      mask TypeOptions popup_animation: Off | On
      mask Display: disp(' ');
  wires:
  DrvBus/1 -> Data for Unreal/2, Dashboard/2(DrvBus)
  VehBus/1 -> Data for Unreal/1, Dashboard/1(VehBus)
  Data for Unreal/1 -> Bus Creator/1, Unreal/1("xyz ")  "xyz"
  Data for Unreal/2 -> Bus Creator/2, Unreal/2("rpy ")  "rpy"
  Data for Unreal/3 -> Bus Creator/3, Unreal/3("ws ")  "ws"
  Data for Unreal/4 -> Bus Creator/4, Unreal/4("aCamber ")  "aCamber"
  Data for Unreal/5 -> Bus Creator/5, Unreal/5("aSteerWheel ")  "aSteerWheel"
  Bus Creator/1 -> Terminator/1  "Unreal_Timeseries"

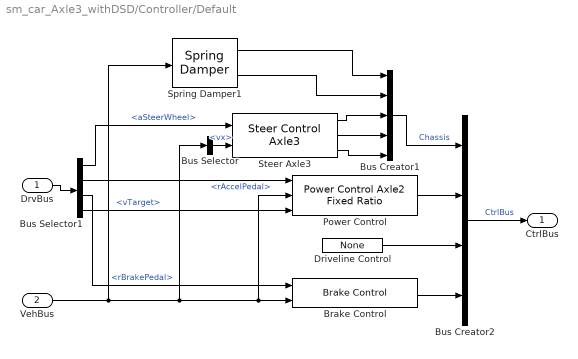
== system sm_car_Axle3_withDSD/Controller/Default ==
  DrvBus : Inport
  VehBus : Inport  Port=2
  Brake Control : Brake_Control/Brake Control  VariantControl=Variant1  LabelModeActiveChoice=Pedal  popup_brake_control=Pedal  abs_tire_radiusF=Vehicle.Chassis.TireA1.tire_radius.Value  abs_tire_radiusR=Vehicle.Chassis.TireA2.tire_radius.Value
      settings: AttributesFormatString=%<ActiveVariant>
  Bus Creator1 : BusCreator  Inputs=5
  Bus Creator2 : BusCreator  Inputs=4
  Bus Selector : BusSelector  OutputSignals=Chassis.Body.CG.vx
  Bus Selector1 : BusSelector  OutputSignals=aSteerWheel,rAccelPedal,rBrakePedal,Reference.vTarget
  Driveline Control : Driveline_Control_Axle2_None/None  SystemSampleTime=-1  VariantActivationTime=update diagram  Latency=0  AutoFrameSizeCalculation=off
  Power Control : Power_Control_Axle2_FixedRatio/Power Control Axle2 Fixed Ratio  trq_max=3000  trq_ratio_front=0.5  trq_rate_up=1000  trq_rate_down=-5000
  Spring Damper1 : Vehicle_Inputs/Control Bus Axle3/Spring Damper  SystemSampleTime=-1  VariantActivationTime=update diagram  Latency=0  AutoFrameSizeCalculation=off
  Steer Axle3 : Steer_Control_Axle3/Steer Control Axle3  nSteerA2=Control.Default.Steer.steer_ratio_axle2  nSteerA3=Control.Default.Steer.steer_ratio_axle3
  CtrlBus : Outport  VectorParamsAs1DForOutWhenUnconnected=off
  wires:
  DrvBus/1 -> Bus Selector1/1
  Bus Creator2/1 -> CtrlBus/1  "CtrlBus"
  Bus Selector1/3 -> Brake Control/1  "<rBrakePedal>"
  Bus Selector1/2 -> Power Control/1  "<rAccelPedal>"
  Steer Axle3/2 -> Bus Creator1/4
  Power Control/1 -> Bus Creator2/2
  Driveline Control/1 -> Bus Creator2/3
  Steer Axle3/1 -> Bus Creator1/3
  Bus Creator1/1 -> Bus Creator2/1  "Chassis"
  Brake Control/1 -> Bus Creator2/4
  Spring Damper1/1 -> Bus Creator1/1
  VehBus/1 -> Spring Damper1/1, Power Control/2, Brake Control/2, Bus Selector/1
  Spring Damper1/2 -> Bus Creator1/2
  Steer Axle3/3 -> Bus Creator1/5
  Bus Selector1/1 -> Steer Axle3/1  "<aSteerWheel>"
  Bus Selector/1 -> Steer Axle3/2  "<vx>"
  Bus Selector1/4 -> Power Control/3  "<vTarget>"

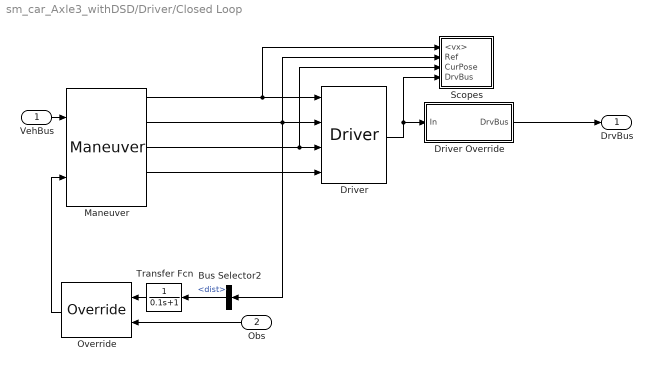
== system sm_car_Axle3_withDSD/Driver/Closed Loop ==
  VehBus : Inport
  Obs : Inport  Port=2
  Bus Selector2 : BusSelector  OutputSignals=dist
  Driver : Driver_Long_Lateral/Driver  Driver=Driver
  Driver Override : Subsystem  Variant=on  VariantControlMode=label  VariantControl=Choice  LabelModeActiveChoice=None  mask{popup_driver_override=None}
      mask prompts: popup_driver_override "Driver Override"
      mask init:
      | curblk = gcb;
      | 
      | set_param(curblk,'LabelModeActiveChoice',get_param(curblk,'popup_driver_override'));
      mask TypeOptions popup_driver_override: None | Override
  Maneuver : Maneuver_Get_Pose/Maneuver  Maneuver=Maneuver  popup_window=No
  Override : Driver_Override/Override  VariantControl=Variant1  LabelModeActiveChoice=None  popup_override_type=None
      settings: AttributesFormatString=%<LabelModeActiveChoice>
  Scopes : Subsystem
  Transfer Fcn : TransferFcn  Denominator=[0.1 1]
  DrvBus : Outport  VectorParamsAs1DForOutWhenUnconnected=off
  wires:
  Transfer Fcn/1 -> Override/1
  Bus Selector2/1 -> Transfer Fcn/1  "<dist>"
  Obs/1 -> Override/2
  Driver Override/1(DrvBus) -> DrvBus/1
  VehBus/1 -> Maneuver/1
  Driver/1 -> Driver Override/1(In), Scopes/4(DrvBus)
  Maneuver/4 -> Driver/4
  Maneuver/1 -> Scopes/1(<vx>), Driver/1
  Maneuver/3 -> Scopes/3(CurPose), Driver/3
  Maneuver/2 -> Bus Selector2/1, Scopes/2(Ref), Driver/2
  Override/1 -> Maneuver/2

== system sm_car_Axle3_withDSD/Driver/Interactive ==
  VehBus : Inport
  Obs : Inport  Port=2
  Driver Inputs Xbox : Driver_Gamepad_Xbox/Gamepad Xbox/Driver Inputs Xbox  SystemSampleTime=-1  VariantActivationTime=update diagram  Latency=0  AutoFrameSizeCalculation=off
  Pace Car : Subsystem  Variant=on  VariantControlMode=label  VariantControl=Variant1  LabelModeActiveChoice=None  mask{popup_pace_car=None}
      mask prompts: popup_pace_car "Pace Car"
      mask init:
      | set_param(gcb,'LabelModeActiveChoice',get_param(gcb,'popup_pace_car'));
      settings: AttributesFormatString=%<popup_pace_car>
      mask TypeOptions popup_pace_car: None | Show
      mask Display: disp(' ');
  Terminator1 : Terminator
  DrvBus : Outport  VectorParamsAs1DForOutWhenUnconnected=off
  wires:
  Obs/1 -> Terminator1/1
  VehBus/1 -> Pace Car/1("VehBus ")
  Driver Inputs Xbox/1 -> DrvBus/1

== system sm_car_Axle3_withDSD/Driver/Open Loop ==
  VehBus : Inport
  Obs : Inport  Port=2
  Open Loop : Driver_Open_Loop/Open Loop  Maneuver=Maneuver
  Terminator : Terminator
  Terminator1 : Terminator
  DrvBus : Outport  VectorParamsAs1DForOutWhenUnconnected=off
  wires:
  Obs/1 -> Terminator1/1
  VehBus/1 -> Terminator/1
  Open Loop/1 -> DrvBus/1

== system sm_car_Axle3_withDSD/Road/Input fWindCar ==
  Bus Creator1 : BusCreator  Inputs=3
  Demux : Demux  Outputs=3
  Step : Step  Time=dWind  After=fWind  SampleTime=0
  Step1 : Step  Time=dWind+tWind  After=fWind  SampleTime=0
  Sum : Sum  Inputs=|+-
  fWind : Outport  VectorParamsAs1DForOutWhenUnconnected=off
  wires:
  Demux/2 -> Bus Creator1/2  "fy"
  Demux/1 -> Bus Creator1/1  "fx"
  Demux/3 -> Bus Creator1/3  "fz"
  Bus Creator1/1 -> fWind/1
  Step/1 -> Sum/1
  Step1/1 -> Sum/2
  Sum/1 -> Demux/1

== system sm_car_Axle3_withDSD/Road/Input fWindTrailer ==
  Bus Creator1 : BusCreator  Inputs=3
  Demux : Demux  Outputs=3
  Scope : Scope
  Step : Step  Time=dWind  After=fWind  SampleTime=0
  Step1 : Step  Time=dWind+tWind  After=fWind  SampleTime=0
  Sum : Sum  Inputs=|+-
  fWind : Outport  VectorParamsAs1DForOutWhenUnconnected=off
  wires:
  Bus Creator1/1 -> fWind/1
  Demux/3 -> Bus Creator1/3  "fz"
  Demux/1 -> Bus Creator1/1  "fx"
  Demux/2 -> Bus Creator1/2  "fy"
  Sum/1 -> Scope/1, Demux/1  "fxyz"
  Step1/1 -> Sum/2
  Step/1 -> Sum/1
